simulink model "parrotMinidroneCompetition"  (R2026a)
settings: Solver=ode3  StartTime=0  StopTime=TFinal  FixedStep=Ts
values from neighbouring files (symbols this model uses):
  sensorCalibrationData = [0.09 -0.06 -9.473 -0.0095 -0.0075 0.0015 101270.95 0.2]    [sensorCalibration.mat]
undefined symbols (not defined in the file or in its folder): Command, ft, init, m, Rec, s, SDTV, Sensors, Sim3dSensor, States, takeOffDuration, Ts, Vehicle
libraries: simulink x16, sim3dlib x5, aerolibconvert2 x4, slpidlib x4, SignalEditorBlockLib x2, environmentLibrary x2, visionconversions x2, visiongeotforms x2, aerolibanimutils x1, aerolibnav x1
(part 1 of 2)
settings Model: ExtModeTrigDuration=80  Creator=The MathWorks, Inc.  LastModifiedBy=khade
settings DebuggingCC: MultiTaskRateTransMsg=warning  ParameterPrecisionLossMsg=none  PregeneratedLibrarySubsystemCodeDiagnostic=none  SubsystemReferenceDiagnosticForUnitTest=warning
settings HardwareCC: ProdLargestAtomicInteger=Long  ProdHWDeviceType=ARM Compatible->ARM 9  UseEmbeddedCoderFeatures=off  UseSimulinkCoderFeatures=off
settings RTWCC: SystemTargetFile=ert.tlc  GenerateReport=on  Toolchain=Sourcery G++ Lite GNU Toolchain for Drones  IncludeHyperlinkInReport=on  LaunchReport=on  GenerateTraceInfo=on  GenerateTraceReport=on  GenerateTraceReportSl=on  GenerateTraceReportSf=on  GenerateTraceReportEml=on  Description=Embedded Coder
settings ERTTargetCC: DynamicArrayContainerType=coder::array

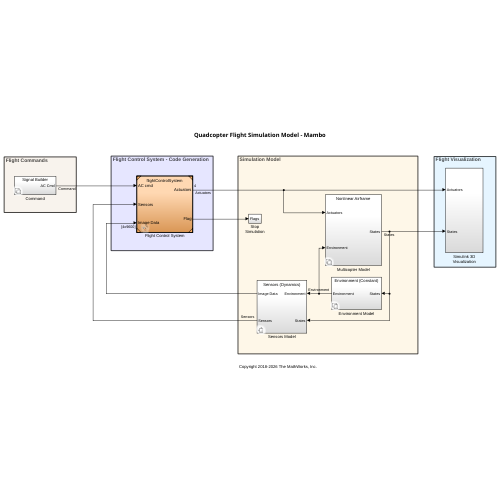
[thumbnail: Simulink's stored preview of the top-level diagram]
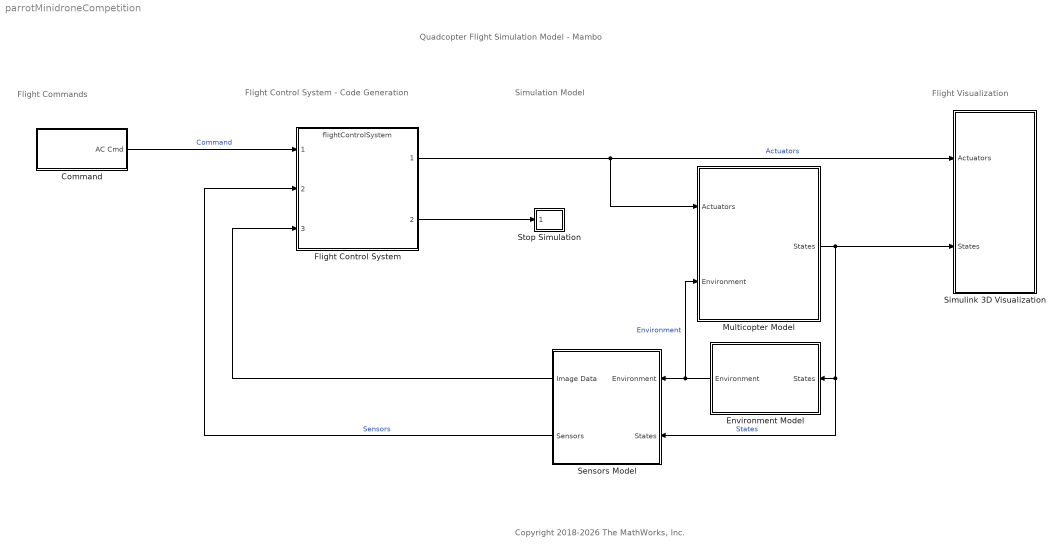
== system parrotMinidroneCompetition ==
  note: Flight Visualization
  note: Simulation Model
  note: Flight Control System - Code Generation
  note: Flight Commands
  note: Quadcopter Flight Simulation Model - Mambo
  note: Copyright 2018-2026 The MathWorks, Inc.
  Command : Subsystem  Variant=on
  Environment Model : Subsystem  Variant=on
  Flight Control System : ModelReference  ModelNameDialog=flightControlSystem.slx  SimulationMode=Normal  ModelReferenceVersion=12.37
  Multicopter Model : Subsystem  Variant=on
  Sensors Model : Subsystem  Variant=on
  Simulink 3D Visualization : Subsystem
  Stop Simulation : Subsystem
  wires:
  Command/1(AC Cmd) -> Flight Control System/1  "Command"
  Sensors Model/2(Sensors) -> Flight Control System/2  "Sensors"
  Flight Control System/1 -> Multicopter Model/1(Actuators), Simulink 3D Visualization/1(Actuators)  "Actuators"
  Environment Model/1(Environment) -> Sensors Model/1(Environment), Multicopter Model/2(Environment)  "Environment"
  Multicopter Model/1(States) -> Sensors Model/2(States), Environment Model/1(States), Simulink 3D Visualization/2(States)  "States"
  Flight Control System/2 -> Stop Simulation/1(Flags)
  Sensors Model/1(Image Data) -> Flight Control System/3

== system parrotMinidroneCompetition/Command ==
  note: VSS_COMMAND = 0 will select Signal Builder
      | VSS_COMMAND =1 will select Joystick + Signal Builder
      | VSS_COMMAND = 2 will select pre-saved data from .mat file
      | VSS_COMMAND = 3 will select pre-saved data from a spreadsheet
  Data : Subsystem  VariantControl=VSS_COMMAND_PRESAVED
  Joystick : Subsystem  VariantControl=VSS_COMMAND_JOYSTICK
  Signal Builder : Subsystem  VariantControl=VSS_COMMAND_SIGBLDR
  Spreadsheet Data : Subsystem  VariantControl=VSS_COMMAND_SPREADSHEET
  AC Cmd : Outport  OutDataTypeStr=Bus: CommandBus  VectorParamsAs1DForOutWhenUnconnected=off

== system parrotMinidroneCompetition/Environment Model ==
  note: VSS_ENVIRONMENT = 0 will select constant environment variables
      | VSS_ENVIRONMENT = 1 will select environment variables depending on position
  States : Inport  OutDataTypeStr=Bus: StatesBus
  Environment (Constant) : environmentLibrary/Environment (Constant)  SystemSampleTime=-1  VariantControl=VSS_ENVIRONMENT_CST  VariantActivationTime=update diagram  EmptyChoice=off  PassThrough=off  PassThroughVariantControl=(default)  EmptyChoiceVariantControl=(default)  AllowFlexibleInterface=on  Latency=0  AutoFrameSizeCalculation=off
  Environment (Variable) : environmentLibrary/Environment (Variable)  SystemSampleTime=-1  VariantControl=VSS_ENVIRONMENT_VARIABLE  VariantActivationTime=update diagram  EmptyChoice=off  PassThrough=off  PassThroughVariantControl=(default)  EmptyChoiceVariantControl=(default)  AllowFlexibleInterface=on  Latency=0  AutoFrameSizeCalculation=off
  Environment : Outport  OutDataTypeStr=Bus: EnvironmentBus  VectorParamsAs1DForOutWhenUnconnected=off

== system parrotMinidroneCompetition/Multicopter Model ==
  note: VSS_VEHICLE = 0 will select linear airframe
      | VSS_VEHICLE = 1 will select nonlnear airframe
  Actuators : Inport
  Environment : Inport  Port=2  OutDataTypeStr=Bus: EnvironmentBus
  Linear Airframe : ModelReference  ModelNameDialog=linearAirframe.slx  SimulationMode=Normal  VariantControl=VSS_VEHICLE_LINEAR  ModelReferenceVersion=17.0
  Nonlinear Airframe : ModelReference  ModelNameDialog=nonlinearAirframe.slx  SimulationMode=Normal  VariantControl=VSS_VEHICLE_NONLINEAR  ModelReferenceVersion=17.1
  States : Outport  OutDataTypeStr=Bus: StatesBus  VectorParamsAs1DForOutWhenUnconnected=off

== system parrotMinidroneCompetition/Sensors Model ==
  note: VSS_SENSORS = 0 will select feedthrough sensors
      | VSS_SENSORS = 1 will select dynamics sensors with noise
  Environment : Inport
  States : Inport  Port=2
  Sensors (Dynamics) : Subsystem  TreatAsAtomicUnit=on  VariantControl=VSS_SENSORS_DYNAMICS
  Sensors (Feedthrough) : Subsystem  TreatAsAtomicUnit=on  VariantControl=VSS_SENSORS_FEEDTHROUGH
  Image Data : Outport  VectorParamsAs1DForOutWhenUnconnected=off
  Sensors : Outport  Port=2  VectorParamsAs1DForOutWhenUnconnected=off

== system parrotMinidroneCompetition/Simulink 3D Visualization ==
  Actuators : Inport
  States : Inport  Port=2
  Extract Flight Instruments : Subsystem
  Simulink 3D : Subsystem  VariantControl=VSS_VISUALIZATION_SL3D
      mask init:
      | visualizationFlightGearVars;
  wires:
  Actuators/1 -> Extract Flight Instruments/1(Actuators), Simulink 3D/2(Actuators)
  States/1 -> Extract Flight Instruments/2(States), Simulink 3D/1(States)

== system parrotMinidroneCompetition/Stop Simulation ==
  Flags : Inport  OutDataTypeStr=uint8
  Compare To Zero : simulink/Logic and Bit Operations/Compare To Zero  relop=>  OutDataTypeStr=boolean
  Flag has been triggered : Assertion
  Logical Operator : Logic  Operator=NOT  AllPortsSameDT=off  OutDataTypeStr=boolean
  wires:
  Flags/1 -> Compare To Zero/1
  Logical Operator/1 -> Flag has been triggered/1
  Compare To Zero/1 -> Logical Operator/1

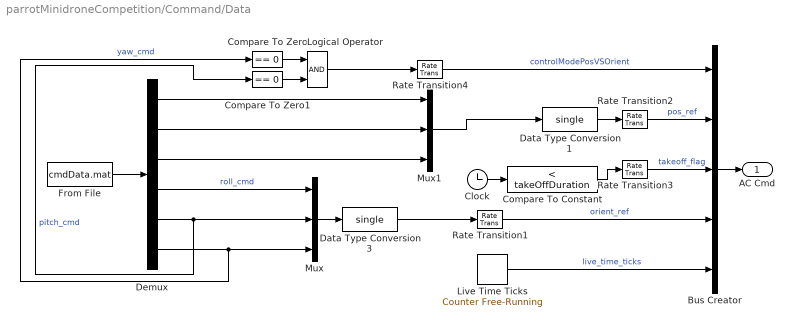
== system parrotMinidroneCompetition/Command/Data ==
  Bus Creator : BusCreator  Inputs=5  OutDataTypeStr=Bus: CommandBus  NonVirtualBus=on
  Clock : Clock
  Compare To Constant : simulink/Logic and Bit Operations/Compare To Constant  relop=<  const=takeOffDuration  OutDataTypeStr=boolean
  Compare To Zero : simulink/Logic and Bit Operations/Compare To Zero  relop===  OutDataTypeStr=boolean
  Compare To Zero1 : simulink/Logic and Bit Operations/Compare To Zero  relop===  OutDataTypeStr=boolean
  Data Type Conversion1 : DataTypeConversion  OutDataTypeStr=single  SaturateOnIntegerOverflow=off  RndMeth=Floor
  Data Type Conversion3 : DataTypeConversion  OutDataTypeStr=single  SaturateOnIntegerOverflow=off  RndMeth=Floor
  Demux : Demux  Outputs=6
  From File : FromFile  FileName=cmdData.mat  SampleTime=Ts
  Live Time Ticks : simulink/Sources/Counter Free-Running  NumBits=32  tsamp=Ts
  Logical Operator : Logic  AllPortsSameDT=off  OutDataTypeStr=boolean
  Mux : Mux  Inputs=3
  Mux1 : Mux  Inputs=3
  Rate Transition{1..4} (4 alike) : RateTransition  OutPortSampleTime=Ts
  AC Cmd : Outport  OutDataTypeStr=Bus: CommandBus  VectorParamsAs1DForOutWhenUnconnected=off
  wires:
  Demux/4 -> Mux/1  "roll_cmd"
  Demux/5 -> Mux/2, Compare To Zero1/1  "pitch_cmd"
  Demux/6 -> Compare To Zero/1, Mux/3  "yaw_cmd"
  From File/1 -> Demux/1
  Logical Operator/1 -> Rate Transition4/1
  Rate Transition1/1 -> Bus Creator/4  "orient_ref"
  Rate Transition2/1 -> Bus Creator/2  "pos_ref"
  Demux/3 -> Mux1/3
  Mux/1 -> Data Type Conversion3/1
  Data Type Conversion1/1 -> Rate Transition2/1
  Demux/1 -> Mux1/1
  Compare To Zero1/1 -> Logical Operator/2
  Compare To Zero/1 -> Logical Operator/1
  Mux1/1 -> Data Type Conversion1/1
  Clock/1 -> Compare To Constant/1
  Rate Transition4/1 -> Bus Creator/1  "controlModePosVSOrient"
  Data Type Conversion3/1 -> Rate Transition1/1
  Demux/2 -> Mux1/2
  Compare To Constant/1 -> Rate Transition3/1
  Rate Transition3/1 -> Bus Creator/3  "takeoff_flag"
  Live Time Ticks/1 -> Bus Creator/5  "live_time_ticks"
  Bus Creator/1 -> AC Cmd/1

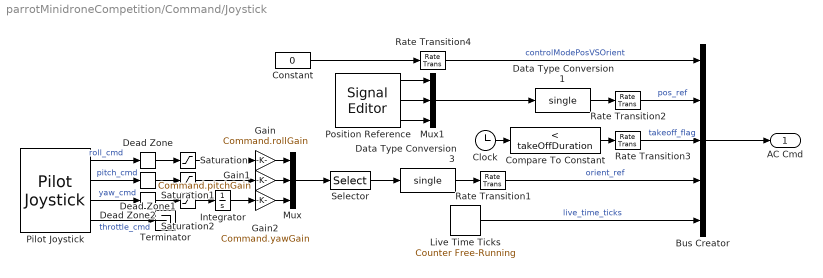
== system parrotMinidroneCompetition/Command/Joystick ==
  Bus Creator : BusCreator  Inputs=5  OutDataTypeStr=Bus: CommandBus  NonVirtualBus=on
  Clock : Clock
  Compare To Constant : simulink/Logic and Bit Operations/Compare To Constant  relop=<  const=takeOffDuration  OutDataTypeStr=boolean
  Constant : Constant  Value=0  OutDataTypeStr=boolean
  Data Type Conversion1 : DataTypeConversion  OutDataTypeStr=single  SaturateOnIntegerOverflow=off  RndMeth=Floor
  Data Type Conversion3 : DataTypeConversion  OutDataTypeStr=single  SaturateOnIntegerOverflow=off  RndMeth=Floor
  Dead Zone : DeadZone  LowerValue=Command.rollDeadZoneStart  UpperValue=Command.rollDeadZoneEnd
  Dead Zone1 : DeadZone  LowerValue=Command.pitchDeadZoneStart  UpperValue=Command.pitchDeadZoneEnd
  Dead Zone2 : DeadZone  LowerValue=Command.yawDeadZoneStart  UpperValue=Command.yawDeadZoneEnd
  Gain : Gain  Gain=Command.rollGain
  Gain1 : Gain  Gain=Command.pitchGain
  Gain2 : Gain  Gain=Command.yawGain
  Integrator : Integrator
  Live Time Ticks : simulink/Sources/Counter Free-Running  NumBits=32  tsamp=Ts
  Mux : Mux  Inputs=3
  Mux1 : Mux  Inputs=3
  Pilot Joystick : aerolibanimutils/Pilot Joystick  JoystickID=Joystick1  OutputConfiguration=FourAxis  SampleTime=Ts
  Position Reference : SignalEditorBlockLib/Signal Editor  FileName=Position_Reference.mat  ActiveScenario=Group_1  ActiveSignal=Z  IsBus=off  OutputBusObjectStr=Bus: BusObject  SampleTime=0  OutputAfterFinalValue=Extrapolation  Unit=inherit  PreserveSignalName=on  ApplySigPropsToAllScenarios=on  ApplySigPropsToAllSignals=off  SignalPropertySource=Dialog parameters
  Rate Transition{1..4} (4 alike) : RateTransition  OutPortSampleTime=Ts
  Saturation : Saturate  UpperLimit=Command.rollSatUpper  LowerLimit=Command.rollSatLower
  Saturation1 : Saturate  UpperLimit=Command.pitchSatUpper  LowerLimit=Command.pitchSatLower
  Saturation2 : Saturate  UpperLimit=Command.yawSatUpper  LowerLimit=Command.yawSatLower
  Selector : Selector  InputPortWidth=3  IndexOptions=Index vector (dialog)  Indices=[3 2 1]  OutputSizes=1
  Terminator : Terminator
  AC Cmd : Outport  OutDataTypeStr=Bus: CommandBus  VectorParamsAs1DForOutWhenUnconnected=off
  wires:
  Pilot Joystick/4 -> Terminator/1  "throttle_cmd"
  Pilot Joystick/1 -> Dead Zone/1  "roll_cmd"
  Bus Creator/1 -> AC Cmd/1
  Constant/1 -> Rate Transition4/1
  Rate Transition1/1 -> Bus Creator/4  "orient_ref"
  Rate Transition2/1 -> Bus Creator/2  "pos_ref"
  Position Reference/3 -> Mux1/3
  Mux/1 -> Selector/1
  Data Type Conversion1/1 -> Rate Transition2/1
  Position Reference/1 -> Mux1/1
  Mux1/1 -> Data Type Conversion1/1
  Compare To Constant/1 -> Rate Transition3/1
  Clock/1 -> Compare To Constant/1
  Rate Transition4/1 -> Bus Creator/1  "controlModePosVSOrient"
  Data Type Conversion3/1 -> Rate Transition1/1
  Pilot Joystick/2 -> Dead Zone1/1  "pitch_cmd"
  Position Reference/2 -> Mux1/2
  Rate Transition3/1 -> Bus Creator/3  "takeoff_flag"
  Live Time Ticks/1 -> Bus Creator/5  "live_time_ticks"
  Selector/1 -> Data Type Conversion3/1
  Dead Zone/1 -> Saturation/1
  Saturation/1 -> Gain/1
  Gain/1 -> Mux/1
  Dead Zone1/1 -> Saturation1/1
  Saturation1/1 -> Gain1/1
  Gain1/1 -> Mux/2
  Dead Zone2/1 -> Saturation2/1
  Saturation2/1 -> Integrator/1
  Gain2/1 -> Mux/3
  Pilot Joystick/3 -> Dead Zone2/1  "yaw_cmd"
  Integrator/1 -> Gain2/1

== system parrotMinidroneCompetition/Command/Signal Builder ==
  Bus Creator : BusCreator  Inputs=5  OutDataTypeStr=Bus: CommandBus  NonVirtualBus=on
  Clock : Clock
  Compare To Constant : simulink/Logic and Bit Operations/Compare To Constant  relop=<  const=takeOffDuration  OutDataTypeStr=boolean
  Compare To Zero : simulink/Logic and Bit Operations/Compare To Zero  relop===  OutDataTypeStr=boolean
  Compare To Zero1 : simulink/Logic and Bit Operations/Compare To Zero  relop===  OutDataTypeStr=boolean
  Data Type Conversion1 : DataTypeConversion  OutDataTypeStr=single  SaturateOnIntegerOverflow=off  RndMeth=Floor
  Data Type Conversion3 : DataTypeConversion  OutDataTypeStr=single  SaturateOnIntegerOverflow=off  RndMeth=Floor
  Live Time Ticks : simulink/Sources/Counter Free-Running  NumBits=32  tsamp=Ts
  Logical Operator : Logic  AllPortsSameDT=off  OutDataTypeStr=boolean
  Mux : Mux  Inputs=3
  Mux1 : Mux  Inputs=3
  Position/Attitude Reference : SignalEditorBlockLib/Signal Editor  FileName=Position_Attitude_Reference.mat  ActiveScenario=Group_1  ActiveSignal=Roll  IsBus=off  OutputBusObjectStr=Bus: BusObject  SampleTime=0  OutputAfterFinalValue=Extrapolation  Unit=inherit  PreserveSignalName=on  ApplySigPropsToAllScenarios=on  ApplySigPropsToAllSignals=off  SignalPropertySource=Dialog parameters
  Rate Transition{1..4} (4 alike) : RateTransition  OutPortSampleTime=Ts
  AC Cmd : Outport  OutDataTypeStr=Bus: CommandBus  VectorParamsAs1DForOutWhenUnconnected=off
  wires:
  Bus Creator/1 -> AC Cmd/1
  Position/Attitude Reference/6 -> Compare To Zero/1, Mux/3  "roll_cmd"
  Position/Attitude Reference/5 -> Mux/2, Compare To Zero1/1  "pitch_cmd"
  Position/Attitude Reference/4 -> Mux/1  "yaw_cmd"
  Mux/1 -> Data Type Conversion3/1
  Data Type Conversion3/1 -> Rate Transition1/1
  Rate Transition1/1 -> Bus Creator/4  "orient_ref"
  Compare To Zero/1 -> Logical Operator/1
  Compare To Zero1/1 -> Logical Operator/2
  Logical Operator/1 -> Rate Transition4/1
  Rate Transition4/1 -> Bus Creator/1  "controlModePosVSOrient"
  Position/Attitude Reference/1 -> Mux1/1
  Position/Attitude Reference/2 -> Mux1/2
  Position/Attitude Reference/3 -> Mux1/3
  Mux1/1 -> Data Type Conversion1/1
  Data Type Conversion1/1 -> Rate Transition2/1
  Rate Transition2/1 -> Bus Creator/2  "pos_ref"
  Clock/1 -> Compare To Constant/1
  Compare To Constant/1 -> Rate Transition3/1
  Rate Transition3/1 -> Bus Creator/3  "takeoff_flag"
  Live Time Ticks/1 -> Bus Creator/5  "live_time_ticks"

== system parrotMinidroneCompetition/Command/Spreadsheet Data ==
  Bus Creator : BusCreator  Inputs=5  OutDataTypeStr=Bus: CommandBus  NonVirtualBus=on
  Clock : Clock
  Compare To Constant : simulink/Logic and Bit Operations/Compare To Constant  relop=<  const=takeOffDuration  OutDataTypeStr=boolean
  Compare To Zero : simulink/Logic and Bit Operations/Compare To Zero  relop===  OutDataTypeStr=boolean
  Compare To Zero1 : simulink/Logic and Bit Operations/Compare To Zero  relop===  OutDataTypeStr=boolean
  Data Type Conversion1 : DataTypeConversion  OutDataTypeStr=single  SaturateOnIntegerOverflow=off  RndMeth=Floor
  Data Type Conversion3 : DataTypeConversion  OutDataTypeStr=single  SaturateOnIntegerOverflow=off  RndMeth=Floor
  From Spreadsheet : FromSpreadsheet  FileName=cmdData.xlsx  SheetName=data  SampleTime=Ts
  Live Time Ticks : simulink/Sources/Counter Free-Running  NumBits=32  tsamp=Ts
  Logical Operator : Logic  AllPortsSameDT=off  OutDataTypeStr=boolean
  Mux : Mux  Inputs=3
  Mux1 : Mux  Inputs=3
  Rate Transition{1..4} (4 alike) : RateTransition  OutPortSampleTime=Ts
  AC Cmd : Outport  OutDataTypeStr=Bus: CommandBus  VectorParamsAs1DForOutWhenUnconnected=off
  wires:
  Bus Creator/1 -> AC Cmd/1
  From Spreadsheet/4 -> Mux/1  "roll_cmd"
  From Spreadsheet/6 -> Mux/3, Compare To Zero/1  "yaw_cmd"
  Logical Operator/1 -> Rate Transition4/1
  Rate Transition1/1 -> Bus Creator/4  "orient_ref"
  Rate Transition2/1 -> Bus Creator/2  "pos_ref"
  From Spreadsheet/3 -> Mux1/3
  Mux/1 -> Data Type Conversion3/1
  Data Type Conversion1/1 -> Rate Transition2/1
  From Spreadsheet/1 -> Mux1/1
  Compare To Zero1/1 -> Logical Operator/2
  Compare To Zero/1 -> Logical Operator/1
  Mux1/1 -> Data Type Conversion1/1
  Compare To Constant/1 -> Rate Transition3/1
  Clock/1 -> Compare To Constant/1
  Rate Transition4/1 -> Bus Creator/1  "controlModePosVSOrient"
  Data Type Conversion3/1 -> Rate Transition1/1
  From Spreadsheet/5 -> Mux/2, Compare To Zero1/1  "pitch_cmd"
  From Spreadsheet/2 -> Mux1/2
  Rate Transition3/1 -> Bus Creator/3  "takeoff_flag"
  Live Time Ticks/1 -> Bus Creator/5  "live_time_ticks"

== system parrotMinidroneCompetition/Sensors Model/Sensors (Dynamics) ==
  States : Inport  OutDataTypeStr=Bus: StatesBus
  Environment : Inport  Port=2  OutDataTypeStr=Bus: EnvironmentBus
  Bus Creator1 : BusCreator  Inputs=3  OutDataTypeStr=Bus: SensorsBus  NonVirtualBus=on
  Bus Creator2 : BusCreator  Inputs=3  OutDataTypeStr=Bus: extraSensorData_t  NonVirtualBus=on
  Constant : Constant  Value=sensorCalibrationData  OutDataTypeStr=single
  Memory1 : Memory  InitialCondition=States  InheritSampleTime=on
  Sensor System : Subsystem
  _DUMMY_FLAG_usePosVIS : Constant  Value=Sensors.dummy.usePosVISFlag  OutDataTypeStr=single  SampleTime=Ts
  _DUMMY_posVIS : Constant  Value=Sensors.dummy.posVISNoVisionAvail  OutDataTypeStr=single  SampleTime=Ts
  Sensors : Outport  OutDataTypeStr=Bus: SensorsBus  VectorParamsAs1DForOutWhenUnconnected=off
  Image Data : Outport  Port=2  VectorParamsAs1DForOutWhenUnconnected=off
  wires:
  Constant/1 -> Bus Creator1/3  "SensorCalibration"
  Memory1/1 -> Sensor System/1(States)
  Bus Creator2/1 -> Bus Creator1/1  "VisionSensors"
  Bus Creator1/1 -> Sensors/1
  States/1 -> Memory1/1
  Environment/1 -> Sensor System/2(Environment)
  _DUMMY_FLAG_usePosVIS/1 -> Bus Creator2/3  "usePosVIS_flag"
  _DUMMY_posVIS/1 -> Bus Creator2/2  "posVIS_data"
  Sensor System/1(opticalFlow_data) -> Bus Creator2/1  "opticalFlow_data"
  Sensor System/2(sensordata_data) -> Bus Creator1/2  "HALSensors"
  Sensor System/3(camera_data) -> Image Data/1

== system parrotMinidroneCompetition/Sensors Model/Sensors (Feedthrough) ==
  States : Inport  OutDataTypeStr=Bus: StatesBus
  Environment : Inport  Port=2  OutDataTypeStr=Bus: EnvironmentBus
  Bus Creator1 : BusCreator  Inputs=3  OutDataTypeStr=Bus: SensorsBus  NonVirtualBus=on
  Bus Creator2 : BusCreator  Inputs=3  OutDataTypeStr=Bus: extraSensorData_t  NonVirtualBus=on
  Constant1 : Constant  Value=sensorCalibrationData  OutDataTypeStr=single
  Memory : Memory  InitialCondition=States  InheritSampleTime=on
  Sensor System : Subsystem
  _DUMMY_FLAG_usePosVIS : Constant  Value=Sensors.dummy.usePosVISFlag  OutDataTypeStr=single
  _DUMMY_posVIS : Constant  Value=Sensors.dummy.posVISNoVisionAvail  OutDataTypeStr=single
  Sensors : Outport  OutDataTypeStr=Bus: SensorsBus  VectorParamsAs1DForOutWhenUnconnected=off
  Image Data : Outport  Port=2  VectorParamsAs1DForOutWhenUnconnected=off
  wires:
  Constant1/1 -> Bus Creator1/3  "SensorCalibration"
  Memory/1 -> Sensor System/1(States)
  Sensor System/2(sensordata_data) -> Bus Creator1/2  "HALSensors"
  States/1 -> Memory/1
  Environment/1 -> Sensor System/2(Environment)
  Bus Creator1/1 -> Sensors/1
  _DUMMY_FLAG_usePosVIS/1 -> Bus Creator2/3  "usePosVIS_flag"
  Sensor System/1(opticalFlow_data) -> Bus Creator2/1  "opticalFlow_data"
  _DUMMY_posVIS/1 -> Bus Creator2/2  "posVIS_data"
  Bus Creator2/1 -> Bus Creator1/1  "VisionSensors"
  Sensor System/3(camera_data) -> Image Data/1

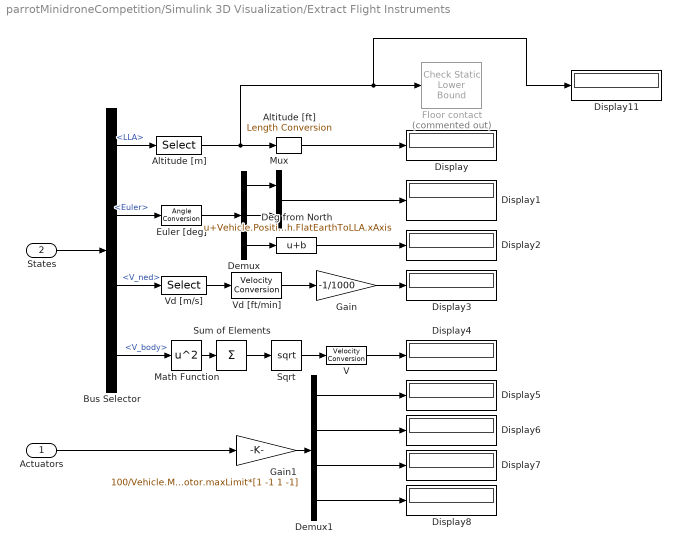
== system parrotMinidroneCompetition/Simulink 3D Visualization/Extract Flight Instruments ==
  Actuators : Inport
  States : Inport  Port=2
  Altitude [ft] : aerolibconvert2/Length Conversion  IU=m  OU=ft
  Altitude [m] : Selector  InputPortWidth=3  IndexOptions=Index vector (dialog)  Indices=[3]  OutputSizes=1
  Bus Selector : BusSelector  OutputSignals=LLA,Euler,V_ned,V_body
  Deg from North : Bias  Bias=Vehicle.PositionOnEarth.FlatEarthToLLA.xAxis  SaturateOnIntegerOverflow=off
  Demux : Demux  Outputs=3
  Demux1 : Demux
  Display{,1..8,11} (10 alike) : Display
  Euler [deg] : aerolibconvert2/Angle Conversion  IU=rad  OU=deg
  Floor contact : simulink/Model Verification/Check Static  Lower Bound  Description=init.posLLA(3) <= u  Commented=on  min=init.posLLA(3)  min_included=on  enabled=on  stopWhenAssertionFail=on  export=off  icon=graphic
  Gain : Gain  Gain=-1/1000
  Gain1 : Gain  Gain=100/Vehicle.Motor.maxLimit*[1 -1 1 -1]
  Math Function : Math  Operator=square  SignedPower=on
  Mux : Mux  Inputs=2
  Sqrt : Sqrt
  Sum of Elements : Sum  Inputs=+
  V : aerolibconvert2/Velocity Conversion  IU=m/s  OU=kts
  Vd [ft/min] : aerolibconvert2/Velocity Conversion  IU=m/s  OU=ft/min
  Vd [m/s] : Selector  InputPortWidth=3  IndexOptions=Index vector (dialog)  Indices=[3]  OutputSizes=1
  wires:
  Bus Selector/1 -> Altitude [m]/1  "<LLA>"
  States/1 -> Bus Selector/1
  Altitude [ft]/1 -> Display/1
  Bus Selector/2 -> Euler [deg]/1  "<Euler>"
  Euler [deg]/1 -> Demux/1
  Demux/1 -> Mux/1
  Demux/2 -> Mux/2
  Mux/1 -> Display1/1
  Deg from North/1 -> Display2/1
  Bus Selector/3 -> Vd [m/s]/1  "<V_ned>"
  Vd [m/s]/1 -> Vd [ft/min]/1
  Vd [ft/min]/1 -> Gain/1
  Gain/1 -> Display3/1
  Math Function/1 -> Sum of Elements/1
  Sum of Elements/1 -> Sqrt/1
  Bus Selector/4 -> Math Function/1  "<V_body>"
  Sqrt/1 -> V/1
  V/1 -> Display4/1
  Gain1/1 -> Demux1/1
  Demux1/1 -> Display5/1
  Demux1/2 -> Display6/1
  Demux1/3 -> Display7/1
  Demux1/4 -> Display8/1
  Actuators/1 -> Gain1/1
  Demux/3 -> Deg from North/1
  Altitude [m]/1 -> Display11/1, Floor contact/1, Altitude [ft]/1

== system parrotMinidroneCompetition/Simulink 3D Visualization/Simulink 3D ==
  States : Inport
  Actuators : Inport  Port=2
  Bus Selector : BusSelector  OutputSignals=Euler,X_ned
  Subsystem : Subsystem
  Subsystem1 : Subsystem
  wires:
  Bus Selector/1 -> Subsystem1/1(Rotation)  "<Euler>"
  Bus Selector/2 -> Subsystem1/2(Translation)  "<X_ned>"
  States/1 -> Bus Selector/1
  Actuators/1 -> Subsystem/1(Actuators)
  Subsystem/1(Position Blade1) -> Subsystem1/3(Blade1.Rotation)
  Subsystem/2(Position Blade 2) -> Subsystem1/4(Blade3.Rotation)
  Subsystem/3(Position Blade 3) -> Subsystem1/5(Blade2.Rotation)
  Subsystem/4(Position Blade 4) -> Subsystem1/6(Blade4.Rotation)

== system parrotMinidroneCompetition/Sensors Model/Sensors (Dynamics)/Sensor System ==
  States : Inport
  Environment : Inport  Port=2
  Camera : Subsystem
  IMU_Pressure : Subsystem
  Rate Transition1 : RateTransition  OutPortSampleTime=Ts
  Rate Transition2 : RateTransition  OutPortSampleTime=Ts
  opticalFlow_data : Outport  VectorParamsAs1DForOutWhenUnconnected=off
  sensordata_data : Outport  Port=2  OutDataTypeStr=Bus: HAL_acquisition_t  VectorParamsAs1DForOutWhenUnconnected=off
  camera_data : Outport  Port=3  VectorParamsAs1DForOutWhenUnconnected=off
  wires:
  Environment/1 -> IMU_Pressure/2(Environment)
  Camera/1(opticalFlow_datout) -> Rate Transition1/1
  IMU_Pressure/1(sensordata_datout) -> Rate Transition2/1
  Rate Transition1/1 -> opticalFlow_data/1
  Rate Transition2/1 -> sensordata_data/1
  States/1 -> Camera/1(states), IMU_Pressure/1(States)
  Camera/2(image_data) -> camera_data/1

== system parrotMinidroneCompetition/Sensors Model/Sensors (Feedthrough)/Sensor System ==
  States : Inport
  Environment : Inport  Port=2
  Camera : Subsystem
  IMU_Pressure : Subsystem
  Rate Transition1 : RateTransition  OutPortSampleTime=Ts
  Rate Transition2 : RateTransition  OutPortSampleTime=Ts
  opticalFlow_data : Outport  VectorParamsAs1DForOutWhenUnconnected=off
  sensordata_data : Outport  Port=2  OutDataTypeStr=Bus: HAL_acquisition_t  VectorParamsAs1DForOutWhenUnconnected=off
  camera_data : Outport  Port=3  VectorParamsAs1DForOutWhenUnconnected=off
  wires:
  Environment/1 -> IMU_Pressure/2(Environment)
  Camera/1(opticalFlow_datout) -> Rate Transition1/1
  IMU_Pressure/1(sensordata_datout) -> Rate Transition2/1
  Rate Transition1/1 -> opticalFlow_data/1
  Rate Transition2/1 -> sensordata_data/1
  States/1 -> Camera/1(states), IMU_Pressure/1(states_datin)
  Camera/2(image_data) -> camera_data/1

== system parrotMinidroneCompetition/Simulink 3D Visualization/Simulink 3D/Subsystem ==
  Actuators : Inport
  Assignment{1..4} (4 alike) : Assignment  DiagnosticForDimensions=Warning  IndexOptions=Index vector (dialog)  Indices=3  OutputSizes=1
  Data Type Conversion : DataTypeConversion  OutDataTypeStr=double  SaturateOnIntegerOverflow=off  RndMeth=Floor
  Demux1 : Demux
  Gain : Gain  Gain=-Vehicle.Motor.commandToW2Gain
  PID Controller{1..4} (4 alike) : slpidlib/PID Controller  Controller=PID  Form=Parallel  TimeDomain=Continuous-time  UseExternalTs=off  SampleTime=-1  IntegratorMethod=Forward Euler  FilterMethod=Forward Euler  ControllerParametersSource=internal  P=0  I=1  UseKiTs=off  D=0  UseExternalDerivativeSource=off  N=100  UseFilter=on  TunerSelectOption=Transfer Function Based (PID Tuner App)  InitialConditionSource=internal  InitialConditionForIntegrator=0  InitialConditionForFilter=0  DifferentiatorICPrevScaledInput=0  ExternalReset=none  TrackingMode=off  Kt=1  LimitOutput=off  SatLimitsSource=internal  UpperSaturationLimit=inf  LowerSaturationLimit=-inf  LinearizeAsGain=on  AntiWindupMode=none  Kb=1  LimitIntegrator=off  UpperIntegratorSaturationLimit=inf  LowerIntegratorSaturationLimit=-inf  POutMin=[]  POutMax=[]  IOutMin=[]  IOutMax=[]  DOutMin=[]  DOutMax=[]  NOutMin=[]  NOutMax=[]  SumOutMin=[]  SumOutMax=[]  SaturationOutMin=[]  SaturationOutMax=[]  PParamMin=[]  PParamMax=[]  IParamMin=[]  IParamMax=[]  DParamMin=[]  DParamMax=[]  NParamMin=[]  NParamMax=[]  KbParamMin=[]  KbParamMax=[]  KtParamMin=[]  KtParamMax=[]  KbOutMin=[]  KbOutMax=[]  KtOutMin=[]  KtOutMax=[]  IntegratorOutMin=[]  IntegratorOutMax=[]  FilterOutMin=[]  FilterOutMax=[]  SumI1OutMin=[]  SumI1OutMax=[]  SumI2OutMin=[]  SumI2OutMax=[]  SumI3OutMin=[]  SumI3OutMax=[]  SumI4OutMin=[]  SumI4OutMax=[]  SumDOutMin=[]  SumDOutMax=[]  DifferentiatorOutMin=[]  DifferentiatorOutMax=[]  FilterDiffOutCoefMin=[]  FilterDiffOutCoefMax=[]  ReciprocalOutMin=[]  ReciprocalOutMax=[]  SumDenOutMin=[]  SumDenOutMax=[]  SumNumOutMin=[]  SumNumOutMax=[]  DivideOutMin=[]  DivideOutMax=[]  UdiffTsProdOutMin=[]  UdiffTsProdOutMax=[]  NTsProdOutMin=[]  NTsProdOutMax=[]  UintegralTsProdOutMin=[]  UintegralTsProdOutMax=[]  UngainTsProdOutMin=[]  UngainTsProdOutMax=[]  ClampingZeroOutDataTypeStr=Inherit: Inherit via back propagation  ClampingZeroOutMin=[]  ClampingZeroOutMax=[]  FilterDenConstantOutDataTypeStr=Inherit: Inherit via back propagation  FilterDenConstantOutMin=[]  FilterDenConstantOutMax=[]  PCopyOutDataTypeStr=Inherit: Inherit via back propagation  PCopyOutMin=[]  PCopyOutMax=[]  NCopyOutDataTypeStr=Inherit: Inherit via back propagation  NCopyOutMin=[]  NCopyOutMax=[]  IntegratorContinuousStateAttributes=''  IntegratorStateMustResolveToSignalObject=off  IntegratorRTWStateStorageClass=Auto  FilterContinuousStateAttributes=''  FilterStateMustResolveToSignalObject=off  FilterRTWStateStorageClass=Auto  ParallelPVariant=InternalParameters  IdealPVariant=Disabled  IVariant=InternalParameters  DVariant=InternalParameters  IntegratorVariant=Continuous  SatVariant=Disabled  AWVariant=Passthrough  PCopyVariant=Disabled  TRVariant=Disabled  FdbkBlocksVariant=Forward  IdealPFdbkVariant=Disabled  SatFdbkVariant=Disabled  DerivativeFilterVariant=ContFilter  NVariant=InternalParameters  NCopyVariant=Disabled  FilterICVariant=InternalICsFilter  IntegratorICVariant=InternalICs  ExternalResetVariant=Disabled  TRSumVariant=Passthrough  SumFdbkVariant=Disabled  SumVariant=Sum_PID  TsampFilterVariant=InternalTs  TsampNgainVariant=Passthrough  TsampIntegralVariant=Disabled_SignalSpec  ExternalSaturationOutDataTypeStr=Inherit: Same as second input  DerivativeSourceVariant=ErrorSignal  PreIntVariant=InternalPreInt
  Propeller Initial Rotation : Constant  Value=[0 0 -pi/2]  VectorParams1D=off
  Visualization Gain : Gain  Gain=.0001
  Position Blade1 : Outport  VectorParamsAs1DForOutWhenUnconnected=off
  Position Blade 2 : Outport  Port=2  VectorParamsAs1DForOutWhenUnconnected=off
  Position Blade 3 : Outport  Port=3  VectorParamsAs1DForOutWhenUnconnected=off
  Position Blade 4 : Outport  Port=4  VectorParamsAs1DForOutWhenUnconnected=off
  wires:
  Visualization Gain/1 -> Demux1/1
  Gain/1 -> Visualization Gain/1
  Actuators/1 -> Data Type Conversion/1
  Data Type Conversion/1 -> Gain/1
  PID Controller3/1 -> Assignment3/2
  Propeller Initial Rotation/1 -> Assignment4/1, Assignment2/1, Assignment1/1, Assignment3/1
  Assignment3/1 -> Position Blade1/1
  Demux1/1 -> PID Controller3/1
  Assignment1/1 -> Position Blade 3/1
  PID Controller1/1 -> Assignment1/2
  Demux1/2 -> PID Controller1/1
  Demux1/3 -> PID Controller2/1
  PID Controller2/1 -> Assignment2/2
  Assignment2/1 -> Position Blade 2/1
  Demux1/4 -> PID Controller4/1
  PID Controller4/1 -> Assignment4/2
  Assignment4/1 -> Position Blade 4/1

== system parrotMinidroneCompetition/Simulink 3D Visualization/Simulink 3D/Subsystem1 ==
  Rotation : Inport
  Translation : Inport  Port=2
  Blade1.Rotation : Inport  Port=3
  Blade3.Rotation : Inport  Port=4
  Blade2.Rotation : Inport  Port=5
  Blade4.Rotation : Inport  Port=6
  Arena : sim3dlib/Simulation 3D Actor  Priority=1  ActorName=Sim3dActor1  ParentName=Scene Origin  Operation=Create at setup  InitScriptText=|  SampleTime=-1  Translation=single([0 0 0])  Rotation=single([0 0 0])  Scale=single([1 1 1])  EventsText=|  aMode=5  ActorTag=Sim3dActor1  ActorType=Sim3dActor  ID=1
      InitScriptText=|
      | % Reserved keywords:
      | % - Actor : handle to this actor object
      | % - World : handle to the world object
      | 
      | % Examples:
      | 
      | % Create a primitive geometry (optional)
      | % createShape(Actor, 'box', [1 1 1]);
      | 
      | % Initialize values (optional)
      | % Actor.Physics = true;
      | % Actor.Color = [1 0 0];
      EventsText=|
      | pillar1.BeginOverlapEvent
      | pillar2.BeginOverlapEvent
      | pillar3.BeginOverlapEvent
      | pillar4.BeginOverlapEvent
      | wall.BeginOverlapEvent   
      | wall_2.BeginOverlapEvent 
      | wall_3.BeginOverlapEvent 
      | wall_4.BeginOverlapEvent
  MATLAB Function : MATLAB Function  TreatAsAtomicUnit=on
  MATLAB Function1 : MATLAB Function  TreatAsAtomicUnit=on
  NOT : Logic  Operator=NOT  IconShape=distinctive  AllPortsSameDT=off  OutDataTypeStr=boolean
  OR : Logic  Operator=OR  Inputs=8  IconShape=distinctive  AllPortsSameDT=off  OutDataTypeStr=boolean
  Quadcopter : sim3dlib/Simulation 3D Actor  Priority=1  ActorName=Quadcopter  ParentName=Scene Origin  Operation=Create at setup  InitScriptText=|  SampleTime=-1  Translation=single([0 0 0])  Rotation=single([0 0 0])  Scale=single([1 1 1])  InputsText=|  aMode=5  ActorTag=Quadcopter  ActorType=Sim3dActor  ID=C
      InitScriptText=|
      | fileName = fullfile(fileparts(fileparts(get_param(bdroot,'FileName'))),'support','Quadcopter.mat');
      | Actor.load(fileName);
      | Actor.Mobility=sim3d.utils.MobilityTypes.Movable;
      | World.Actors.QuadBody.Collisions = 0; % Disable Collisions
      | propagate(World.Actors.QuadBody, 'OverlapEventEnabled',true);
      | % World.Actors.QuadBody.Translation = [-1.5 -1 0.05];
      InputsText=|
      | Quadcopter.Translation
      | Quadcopter.Rotation    
      | Blade1.Rotation       
      | Blade3.Rotation       
      | Blade2.Rotation       
      | Blade4.Rotation
  Rate Transition1 : RateTransition
  Rate Transition2 : RateTransition
  Simulation 3D Scene Configuration : sim3dlib/Simulation 3D Scene Configuration  Priority=0  ProjectFormat=Default Scenes  SceneDesc=Empty scene  ProjectName=E:\New folder\toolbox\shared\sim3d_projects\automotive_project_windows\UE\WindowsNoEditor\VehicleSimulation.exe  ScenePath=/Game/Maps/HwStrght  EnableOpenDRIVE=off  vehTagList={'Custom';'Quadcopter';'Scene Origin';'Sim3dActor1'}  vehTag=Quadcopter  AttachedCameraRelativeTranslation=[0 0 1.5]  FreeCameraDefaultInitialTranslation=[-6, 0, 2]  AttachedCameraRelativeRotation=[0 -90 0]  FreeCameraDefaultInitialRotation=[0, -15, 0]  ViewpointName=Custom  FreeCameraInitialTranslation=[2 2 5]  FreeCameraInitialRotation=[0 -90 0]  OpVisEn=off  Ts=.02  EnableWindow=on  EnableRemoteAccess=off  SimulationMode=CoSimulation  SimulateUsing=Interpreted execution  EnableAnimationRecording=off  OverrideDefaultRecording=off  AnimationRecordingFileName=sim3dAnimation.mat  AnimationRecordingInterval=[0 inf]  EnableWeather=off  SunAzimuth=90  SunAltitude=40.0  EnableGeospatialSun=off  Latitude=0  Longitude=0  Date=2023-01-01  Time=10:30:00  GeoTimeZone=-5.0  SunDaylightSaving=off  wind=1  clouds=10  EnableVolumetricClouds=off  CloudCoverage=0  CloudAltitude=6  fog=0  rain=0  RaindropsEffect=off  SnowDensity=0  EnableGeospatial=off  TilesetSource=Earth terrain  UseTrueOrigin=off  OriginHeight=200  OriginLatitude=40.744652  OriginLongitude=-73.988864  MapStyle=Aerial  AdditionalAssetIDs=[]  UseAdvancedSunSky=off  SolarTime=11  TimeZone=-5  Day=21  Month=9  Year=2022  UseDaylightSavingTime=on  DSTStartDay=10  DSTStartMonth=3  DSTEndDay=3  DSTEndMonth=11  DSTSwitchHour=2  sensorTag=MainCamera1  sensorId=1  sensorName=MainCamera1  mountLoc=Origin  offsetFlag=off  tmountOffset=[0, 0, 0]  rmountOffset=[0, 0, 0]  HorizontalResolution=1280  VerticalResolution=720  HorizontalFOV=60  mountPoint=[0 0 0]  mountOrientation=[0 0 0]  aMode=5  ID=1  GeoTrigger=Inactive  ViewNameList={'Custom'}  ViewTranslationList={'[2 2 5]'}  ViewRotationList={'[0 -90 0]'}
      settings: LibrarySourceBlock=sl3dlib/Simulation 3D/Environment/Simulation 3D Scene Configuration
  Stop Simulation : Assertion  AssertionFailFcn=error('The model has stopped as the drone hit the boundary.')
  Terminator : Terminator
  Terminator1 : Terminator
  wires:
  Arena/3 -> OR/2
  Translation/1 -> MATLAB Function1/1(nedCoords)
  Arena/5 -> OR/4
  Arena/1 -> Terminator1/1
  NOT/1 -> Stop Simulation/1
  Rotation/1 -> MATLAB Function/1(nedEuler)
  Quadcopter/1 -> Terminator/1
  Arena/6 -> OR/5
  Arena/2 -> OR/1
  Arena/4 -> OR/3
  Arena/7 -> OR/6
  Arena/8 -> OR/7
  Arena/9 -> OR/8
  MATLAB Function1/1(ue4Coords) -> Rate Transition1/1
  MATLAB Function/1(ue4Euler) -> Rate Transition2/1
  OR/1 -> NOT/1
  Rate Transition1/1 -> Quadcopter/1
  Rate Transition2/1 -> Quadcopter/2
  Blade1.Rotation/1 -> Quadcopter/3
  Blade3.Rotation/1 -> Quadcopter/4
  Blade2.Rotation/1 -> Quadcopter/5
  Blade4.Rotation/1 -> Quadcopter/6

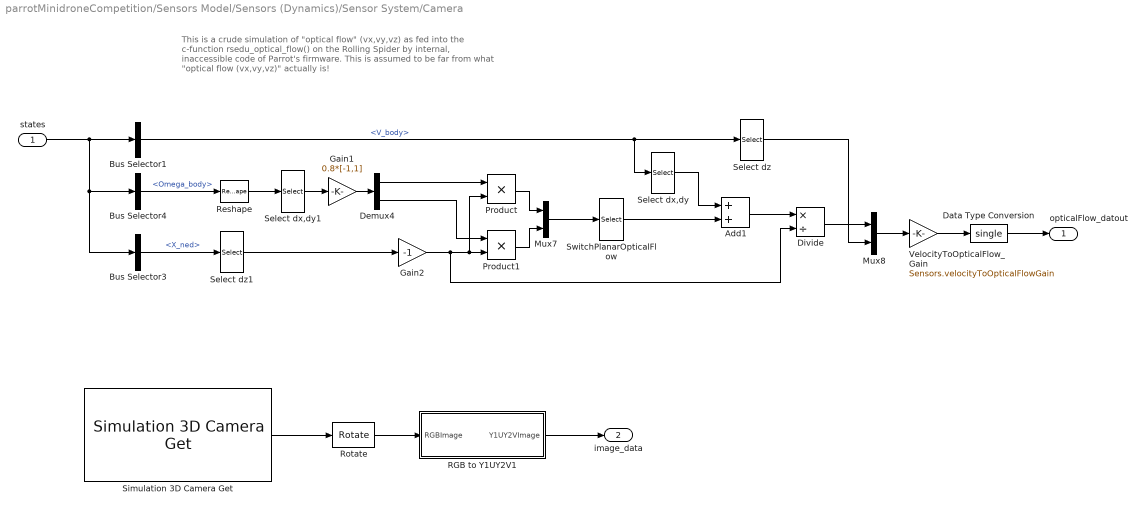
== system parrotMinidroneCompetition/Sensors Model/Sensors (Dynamics)/Sensor System/Camera ==
  note: This is a crude simulation of "optical flow" (vx,vy,vz) as
      | fed into the c-function rsedu_optical_flow() on the Rolling Spider
      | by internal, inaccessible code of Parrot's firmware.
      | This is assumed to be far from what "optical flow (vx,vy,vz)" actually is!
  states : Inport  OutDataTypeStr=Bus: StatesBus
  Add1 : Sum
  Bus Selector1 : BusSelector  OutputSignals=V_body
  Bus Selector3 : BusSelector  OutputSignals=X_ned
  Bus Selector4 : BusSelector  OutputSignals=Omega_body
  Data Type Conversion : DataTypeConversion  OutDataTypeStr=single  SaturateOnIntegerOverflow=off  RndMeth=Floor
  Demux4 : Demux  Outputs=2
  Divide : Product  Inputs=*/
  Gain1 : Gain  Gain=0.8*[-1,1]
  Gain2 : Gain  Gain=-1
  Mux7 : Mux  Inputs=2
  Mux8 : Mux  Inputs=2
  Product : Product
  Product1 : Product
  RGB to Y1UY2V1 : Subsystem
  Reshape : Reshape
  Rotate : visiongeotforms/Rotate  outSizeR=Expanded to fit rotated input image  src_angle=Specify via dialog  unit_angle=Degrees  angle=pi/2  maxAngle=pi  dispImage=Top-left corner  method=Table lookup  fillVal=0  interpMethod=Bilinear  roundingMode=Nearest  overflowMode=on  prodOutputMode=Binary point scaling  prodOutputWordLength=32  prodOutputFracLength=10
  Select dx,dy : Selector  InputPortWidth=3  IndexOptions=Index vector (dialog)  Indices=[1 2]  OutputSizes=1
  Select dx,dy1 : Selector  InputPortWidth=3  IndexOptions=Index vector (dialog)  Indices=[1 2]  OutputSizes=1
  Select dz : Selector  InputPortWidth=3  IndexOptions=Index vector (dialog)  Indices=3  OutputSizes=1
  Select dz1 : Selector  InputPortWidth=3  IndexOptions=Index vector (dialog)  Indices=3  OutputSizes=1
  Simulation 3D Camera Get : sim3dlib/Simulation 3D Camera Get  Priority=1  sensorTag=Sim3dSensor�  sensorId=1  sensorName=Sim3dSensor�  vehTagList={'Quadcopter';'Scene Origin';'Sim3dActor1'}  vehTag=Quadcopter  CoordinateSystem=VRML  mountLoc=Origin  offsetFlag=on  tmountOffset=[0, -0.1, 0]  rmountOffset=[0,deg2rad(-90),deg2rad(90)]  HorizontalResolution=120  VerticalResolution=160  HorizontalFOV=38  SampleTime=0.2  mountPoint=[0 -0.1 0]  mountOrientation=[0 1.5707963267949 -1.5707963267949]  aMode=5  ID=1
      settings: LibrarySourceBlock=sl3dlib/Simulation 3D/Utilities/Simulation 3D Camera Get
  SwitchPlanarOpticalFlow : Selector  InputPortWidth=2  IndexOptions=Index vector (dialog)  Indices=[2 1]  OutputSizes=1
  VelocityToOpticalFlow_Gain : Gain  Gain=Sensors.velocityToOpticalFlowGain
  opticalFlow_datout : Outport  VectorParamsAs1DForOutWhenUnconnected=off
  image_data : Outport  Port=2  VectorParamsAs1DForOutWhenUnconnected=off
  wires:
  SwitchPlanarOpticalFlow/1 -> Add1/2
  Select dz/1 -> Mux8/2
  Bus Selector3/1 -> Select dz1/1  "<X_ned>"
  Mux7/1 -> SwitchPlanarOpticalFlow/1
  Bus Selector4/1 -> Reshape/1  "<Omega_body>"
  VelocityToOpticalFlow_Gain/1 -> Data Type Conversion/1
  Select dx,dy/1 -> Add1/1
  Reshape/1 -> Select dx,dy1/1
  Data Type Conversion/1 -> opticalFlow_datout/1
  Gain2/1 -> Divide/2, Product1/2, Product/2
  Divide/1 -> Mux8/1
  Product1/1 -> Mux7/2
  Select dx,dy1/1 -> Gain1/1
  Simulation 3D Camera Get/1 -> Rotate/1
  Product/1 -> Mux7/1
  RGB to Y1UY2V1/1(Y1UY2VImage) -> image_data/1
  Demux4/1 -> Product/1
  Gain1/1 -> Demux4/1
  Select dz1/1 -> Gain2/1
  Rotate/1 -> RGB to Y1UY2V1/1(RGBImage)
  Bus Selector1/1 -> Select dz/1, Select dx,dy/1  "<V_body>"
  Demux4/2 -> Product1/1
  Mux8/1 -> VelocityToOpticalFlow_Gain/1
  states/1 -> Bus Selector1/1, Bus Selector4/1, Bus Selector3/1
  Add1/1 -> Divide/1

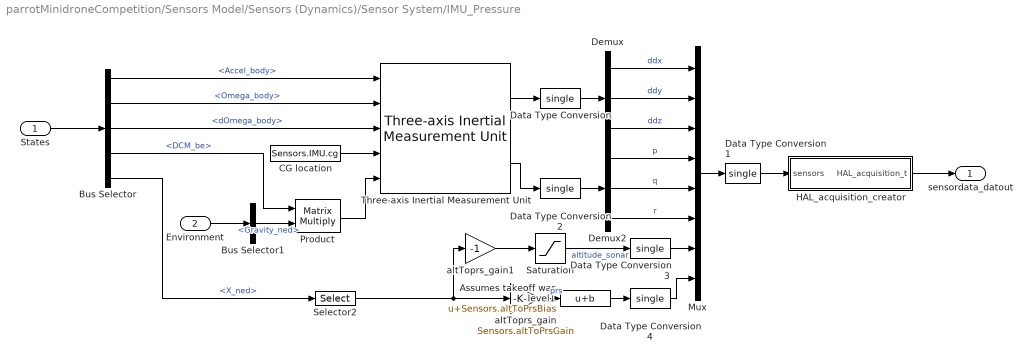
== system parrotMinidroneCompetition/Sensors Model/Sensors (Dynamics)/Sensor System/IMU_Pressure ==
  States : Inport
  Environment : Inport  Port=2
  Assumes takeoff was level1 : Bias  Bias=Sensors.altToPrsBias  SaturateOnIntegerOverflow=off
  Bus Selector : BusSelector  OutputSignals=Accel_body,Omega_body,dOmega_body,DCM_be,X_ned
  Bus Selector1 : BusSelector  OutputSignals=Gravity_ned
  CG location : Constant  Value=Sensors.IMU.cg
  Data Type Conversion{,1..4} (5 alike) : DataTypeConversion  OutDataTypeStr=single  SaturateOnIntegerOverflow=off  RndMeth=Floor
  Demux : Demux  Outputs=3
  Demux2 : Demux  Outputs=3
  HAL_acquisition_creator : Subsystem
  Mux : Mux  Inputs=8
  Product : Product  Multiplication=Matrix(*)
  Saturation : Saturate  UpperLimit=inf  LowerLimit=Sensors.altSensorMin  OutDataTypeStr=single
  Selector2 : Selector  InputPortWidth=3  IndexOptions=Index vector (dialog)  Indices=[3]  OutputSizes=1
  Three-axis Inertial Measurement Unit : aerolibnav/Three-axis Inertial Measurement Unit  units=Metric (MKS)  imu=Sensors.IMU.location  i_Ts=Ts  dtype_a=off  w_a=.7  z_a=.2  a_sf_cc=Sensors.IMU.accScaleCross  a_bias=Sensors.IMU.accBias  a_sat=Sensors.IMU.accLimits  dtype_g=off  w_g=.7  z_g=.2  g_sf_cc=Sensors.IMU.gyroScaleCross  g_bias=Sensors.IMU.gyroBias  g_sens=Sensors.IMU.gyroGBias  g_sat=Sensors.IMU.gyroLimits  i_rand=on  i_seeds=Sensors.IMU.noiseSeeds  i_pow=Sensors.IMU.noisePower
  altToprs_gain : Gain  Gain=Sensors.altToPrsGain  ParamDataTypeStr=single  OutDataTypeStr=single
  altToprs_gain1 : Gain  Gain=-1  ParamDataTypeStr=single  OutDataTypeStr=single
  sensordata_datout : Outport  OutDataTypeStr=Bus: HAL_acquisition_t  VectorParamsAs1DForOutWhenUnconnected=off
  wires:
  altToprs_gain1/1 -> Saturation/1
  Data Type Conversion4/1 -> Mux/8
  Data Type Conversion3/1 -> Mux/7
  Data Type Conversion2/1 -> Demux2/1
  Data Type Conversion/1 -> Demux/1
  Assumes takeoff was level1/1 -> Data Type Conversion4/1
  Bus Selector/5 -> Selector2/1  "<X_ned>"
  States/1 -> Bus Selector/1
  Product/1 -> Three-axis Inertial Measurement Unit/5
  Bus Selector1/1 -> Product/2  "<Gravity_ned>"
  Bus Selector/4 -> Product/1  "<DCM_be>"
  CG location/1 -> Three-axis Inertial Measurement Unit/4
  Bus Selector/3 -> Three-axis Inertial Measurement Unit/3  "<dOmega_body>"
  Environment/1 -> Bus Selector1/1
  Bus Selector/2 -> Three-axis Inertial Measurement Unit/2  "<Omega_body>"
  Bus Selector/1 -> Three-axis Inertial Measurement Unit/1  "<Accel_body>"
  HAL_acquisition_creator/1(HAL_acquisition_t) -> sensordata_datout/1
  Data Type Conversion1/1 -> HAL_acquisition_creator/1(sensors)
  Three-axis Inertial Measurement Unit/2 -> Data Type Conversion2/1
  Three-axis Inertial Measurement Unit/1 -> Data Type Conversion/1
  Mux/1 -> Data Type Conversion1/1
  altToprs_gain/1 -> Assumes takeoff was level1/1  "prs"
  Saturation/1 -> Data Type Conversion3/1  "altitude_sonar"
  Selector2/1 -> altToprs_gain/1, altToprs_gain1/1
  Demux/3 -> Mux/3  "ddz"
  Demux2/3 -> Mux/6  "r"
  Demux/2 -> Mux/2  "ddy"
  Demux/1 -> Mux/1  "ddx"
  Demux2/1 -> Mux/4  "p"
  Demux2/2 -> Mux/5  "q"

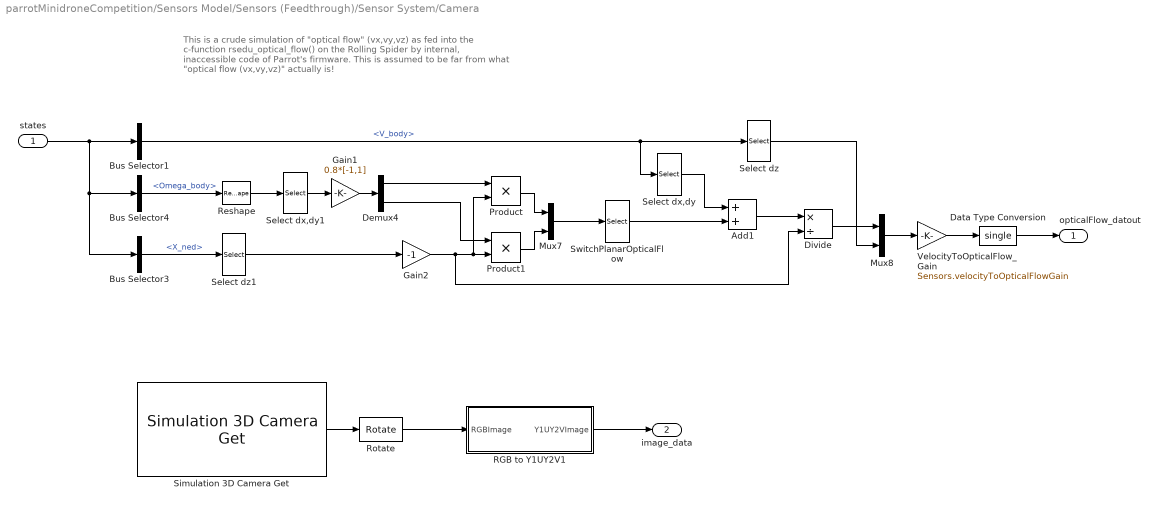
== system parrotMinidroneCompetition/Sensors Model/Sensors (Feedthrough)/Sensor System/Camera ==
  note: This is a crude simulation of "optical flow" (vx,vy,vz) as
      | fed into the c-function rsedu_optical_flow() on the Rolling Spider
      | by internal, inaccessible code of Parrot's firmware.
      | This is assumed to be far from what "optical flow (vx,vy,vz)" actually is!
  states : Inport  OutDataTypeStr=Bus: StatesBus
  Add1 : Sum
  Bus Selector1 : BusSelector  OutputSignals=V_body
  Bus Selector3 : BusSelector  OutputSignals=X_ned
  Bus Selector4 : BusSelector  OutputSignals=Omega_body
  Data Type Conversion : DataTypeConversion  OutDataTypeStr=single  SaturateOnIntegerOverflow=off  RndMeth=Floor
  Demux4 : Demux  Outputs=2
  Divide : Product  Inputs=*/
  Gain1 : Gain  Gain=0.8*[-1,1]
  Gain2 : Gain  Gain=-1
  Mux7 : Mux  Inputs=2
  Mux8 : Mux  Inputs=2
  Product : Product
  Product1 : Product
  RGB to Y1UY2V1 : Subsystem
  Reshape : Reshape
  Rotate : visiongeotforms/Rotate  outSizeR=Expanded to fit rotated input image  src_angle=Specify via dialog  unit_angle=Degrees  angle=pi/2  maxAngle=pi  dispImage=Top-left corner  method=Table lookup  fillVal=0  interpMethod=Bilinear  roundingMode=Nearest  overflowMode=on  prodOutputMode=Binary point scaling  prodOutputWordLength=32  prodOutputFracLength=10
  Select dx,dy : Selector  InputPortWidth=3  IndexOptions=Index vector (dialog)  Indices=[1 2]  OutputSizes=1
  Select dx,dy1 : Selector  InputPortWidth=3  IndexOptions=Index vector (dialog)  Indices=[1 2]  OutputSizes=1
  Select dz : Selector  InputPortWidth=3  IndexOptions=Index vector (dialog)  Indices=3  OutputSizes=1
  Select dz1 : Selector  InputPortWidth=3  IndexOptions=Index vector (dialog)  Indices=3  OutputSizes=1
  Simulation 3D Camera Get : sim3dlib/Simulation 3D Camera Get  Priority=1  sensorTag=Sim3dSensor�  sensorId=3  sensorName=Sim3dSensor�  vehTagList={'Quadcopter';'Scene Origin';'Sim3dActor1'}  vehTag=Quadcopter  CoordinateSystem=VRML  mountLoc=Origin  offsetFlag=on  tmountOffset=[0,-0.1,0]  rmountOffset=[0,deg2rad(-90),deg2rad(90)]  HorizontalResolution=120  VerticalResolution=160  HorizontalFOV=38  SampleTime=0.2  mountPoint=[0 -0.1 0]  mountOrientation=[0 1.5707963267949 -1.5707963267949]  aMode=5  ID=3
      settings: LibrarySourceBlock=sl3dlib/Simulation 3D/Utilities/Simulation 3D Camera Get
  SwitchPlanarOpticalFlow : Selector  InputPortWidth=2  IndexOptions=Index vector (dialog)  Indices=[2 1]  OutputSizes=1
  VelocityToOpticalFlow_Gain : Gain  Gain=Sensors.velocityToOpticalFlowGain
  opticalFlow_datout : Outport  VectorParamsAs1DForOutWhenUnconnected=off
  image_data : Outport  Port=2  VectorParamsAs1DForOutWhenUnconnected=off
  wires:
  SwitchPlanarOpticalFlow/1 -> Add1/2
  Select dz/1 -> Mux8/2
  Bus Selector3/1 -> Select dz1/1  "<X_ned>"
  Mux7/1 -> SwitchPlanarOpticalFlow/1
  Bus Selector4/1 -> Reshape/1  "<Omega_body>"
  VelocityToOpticalFlow_Gain/1 -> Data Type Conversion/1
  Select dx,dy/1 -> Add1/1
  Reshape/1 -> Select dx,dy1/1
  Data Type Conversion/1 -> opticalFlow_datout/1
  Gain2/1 -> Divide/2, Product1/2, Product/2
  Divide/1 -> Mux8/1
  Product1/1 -> Mux7/2
  Select dx,dy1/1 -> Gain1/1
  Product/1 -> Mux7/1
  Demux4/1 -> Product/1
  Gain1/1 -> Demux4/1
  Select dz1/1 -> Gain2/1
  Bus Selector1/1 -> Select dz/1, Select dx,dy/1  "<V_body>"
  Demux4/2 -> Product1/1
  Mux8/1 -> VelocityToOpticalFlow_Gain/1
  states/1 -> Bus Selector1/1, Bus Selector4/1, Bus Selector3/1
  Add1/1 -> Divide/1
  Rotate/1 -> RGB to Y1UY2V1/1(RGBImage)
  RGB to Y1UY2V1/1(Y1UY2VImage) -> image_data/1
  Simulation 3D Camera Get/1 -> Rotate/1

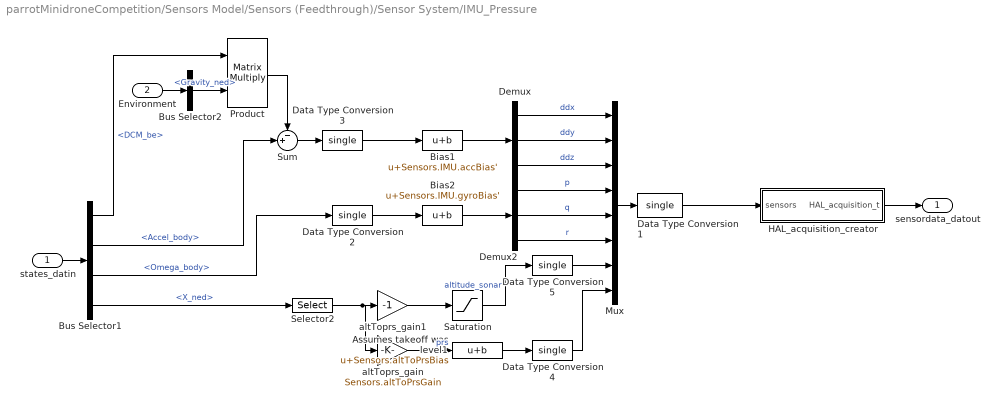
== system parrotMinidroneCompetition/Sensors Model/Sensors (Feedthrough)/Sensor System/IMU_Pressure ==
  states_datin : Inport  OutDataTypeStr=Bus: StatesBus
  Environment : Inport  Port=2
  Assumes takeoff was level1 : Bias  Bias=Sensors.altToPrsBias  SaturateOnIntegerOverflow=off
  Bias1 : Bias  Bias=Sensors.IMU.accBias'  SaturateOnIntegerOverflow=off
  Bias2 : Bias  Bias=Sensors.IMU.gyroBias'  SaturateOnIntegerOverflow=off
  Bus Selector1 : BusSelector  OutputSignals=DCM_be,Accel_body,Omega_body,X_ned
  Bus Selector2 : BusSelector  OutputSignals=Gravity_ned
  Data Type Conversion{1..5} (5 alike) : DataTypeConversion  OutDataTypeStr=single  SaturateOnIntegerOverflow=off  RndMeth=Floor
  Demux : Demux  Outputs=3
  Demux2 : Demux  Outputs=3
  HAL_acquisition_creator : Subsystem
  Mux : Mux  Inputs=8
  Product : Product  Multiplication=Matrix(*)
  Saturation : Saturate  UpperLimit=inf  LowerLimit=Sensors.altSensorMin  OutDataTypeStr=single
  Selector2 : Selector  InputPortWidth=3  IndexOptions=Index vector (dialog)  Indices=[3]  OutputSizes=1
  Sum : Sum  Inputs=-+|
  altToprs_gain : Gain  Gain=Sensors.altToPrsGain  ParamDataTypeStr=single  OutDataTypeStr=single
  altToprs_gain1 : Gain  Gain=-1  ParamDataTypeStr=single  OutDataTypeStr=single
  sensordata_datout : Outport  OutDataTypeStr=Bus: HAL_acquisition_t  VectorParamsAs1DForOutWhenUnconnected=off
  wires:
  Bias2/1 -> Demux2/1
  Bias1/1 -> Demux/1
  Product/1 -> Sum/1
  Bus Selector1/2 -> Sum/2  "<Accel_body>"
  Sum/1 -> Data Type Conversion3/1
  Bus Selector1/1 -> Product/1  "<DCM_be>"
  Bus Selector2/1 -> Product/2  "<Gravity_ned>"
  altToprs_gain1/1 -> Saturation/1
  Data Type Conversion5/1 -> Mux/7
  Data Type Conversion4/1 -> Mux/8
  Data Type Conversion2/1 -> Bias2/1
  Data Type Conversion3/1 -> Bias1/1
  Assumes takeoff was level1/1 -> Data Type Conversion4/1
  Bus Selector1/4 -> Selector2/1  "<X_ned>"
  states_datin/1 -> Bus Selector1/1
  Environment/1 -> Bus Selector2/1
  Bus Selector1/3 -> Data Type Conversion2/1  "<Omega_body>"
  HAL_acquisition_creator/1(HAL_acquisition_t) -> sensordata_datout/1
  Data Type Conversion1/1 -> HAL_acquisition_creator/1(sensors)
  Mux/1 -> Data Type Conversion1/1
  altToprs_gain/1 -> Assumes takeoff was level1/1  "prs"
  Saturation/1 -> Data Type Conversion5/1  "altitude_sonar"
  Selector2/1 -> altToprs_gain1/1, altToprs_gain/1
  Demux/3 -> Mux/3  "ddz"
  Demux2/3 -> Mux/6  "r"
  Demux/2 -> Mux/2  "ddy"
  Demux/1 -> Mux/1  "ddx"
  Demux2/1 -> Mux/4  "p"
  Demux2/2 -> Mux/5  "q"

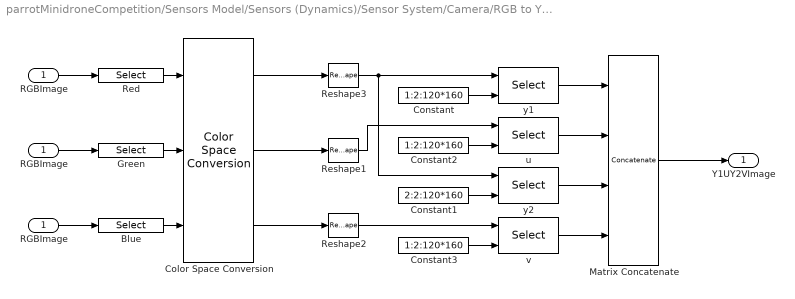
== system parrotMinidroneCompetition/Sensors Model/Sensors (Dynamics)/Sensor System/Camera/RGB to Y1UY2V1 ==
  RGBImage : Inport  OutDataTypeStr=uint8  PortDimensions=[120 160 3]
  " RGBImage " : InportShadow  OutDataTypeStr=uint8  PortDimensions=[120 160 3]
  Blue : Selector  NumberOfDimensions=3  InputPortWidth=3  IndexOptions=Select all,Select all,Index vector (dialog)  Indices=1,1,3  OutputSizes=1,1,1
  Color Space Conversion : visionconversions/Color Space  Conversion  conversion=Obsolete  conversionActive=R'G'B' to Y'CbCr  wp_str=D65  rec=Rec. 601 (SDTV)  sys=1125/60/2:1  imagePorts=Separate color signals
  Constant : Constant  Value=1:2:120*160
  Constant1 : Constant  Value=2:2:120*160
  Constant2 : Constant  Value=1:2:120*160
  Constant3 : Constant  Value=1:2:120*160
  Green : Selector  NumberOfDimensions=3  InputPortWidth=3  IndexOptions=Select all,Select all,Index vector (dialog)  Indices=1,1,2  OutputSizes=1,1,1
  Matrix Concatenate : Concatenate  NumInputs=4  Mode=Multidimensional array
  "RGBImage " : InportShadow  OutDataTypeStr=uint8  PortDimensions=[120 160 3]
  Red : Selector  NumberOfDimensions=3  InputPortWidth=3  IndexOptions=Select all,Select all,Index vector (dialog)  Indices=1,1,1  OutputSizes=1,1,1
  Reshape1 : Reshape  OutputDimensionality=Customize  OutputDimensions=[1,19200]
  Reshape2 : Reshape  OutputDimensionality=Customize  OutputDimensions=[1,19200]
  Reshape3 : Reshape  OutputDimensionality=Customize  OutputDimensions=[1,19200]
  u : Selector  InputPortWidth=120*160  IndexOptions=Index vector (port)  Indices=[1 3]  OutputSizes=1
  v : Selector  InputPortWidth=120*160  IndexOptions=Index vector (port)  Indices=[1 3]  OutputSizes=1
  y1 : Selector  InputPortWidth=120*160  IndexOptions=Index vector (port)  Indices=[1 3]  OutputSizes=1
  y2 : Selector  InputPortWidth=120*160  IndexOptions=Index vector (port)  Indices=[1 3]  OutputSizes=1
  Y1UY2VImage : Outport  OutDataTypeStr=uint8  PortDimensions=[4 9600]  VectorParamsAs1DForOutWhenUnconnected=off
  wires:
  v/1 -> Matrix Concatenate/4
  y1/1 -> Matrix Concatenate/1
  RGBImage/1 -> Green/1
  Red/1 -> Color Space Conversion/1
  Green/1 -> Color Space Conversion/2
  Blue/1 -> Color Space Conversion/3
  Reshape3/1 -> y1/1, y2/1
  Reshape1/1 -> u/1
  Reshape2/1 -> v/1
  Constant/1 -> y1/2
  Constant1/1 -> y2/2
  Constant2/1 -> u/2
  Constant3/1 -> v/2
  Matrix Concatenate/1 -> Y1UY2VImage/1
  u/1 -> Matrix Concatenate/2
  y2/1 -> Matrix Concatenate/3
  " RGBImage "/1 -> Red/1
  "RGBImage "/1 -> Blue/1
  Color Space Conversion/1 -> Reshape3/1
  Color Space Conversion/2 -> Reshape1/1
  Color Space Conversion/3 -> Reshape2/1
